simulink library "lib_highLevelController"  (R2025a)
settings: Solver=VariableStepAuto  StartTime=0.0  StopTime=10.0  RelTol=1e-3
settings Model: Creator=Ruben Rodriguez  LastModifiedBy=gordi
settings RTWCC: GPUComputeCapability=3.5

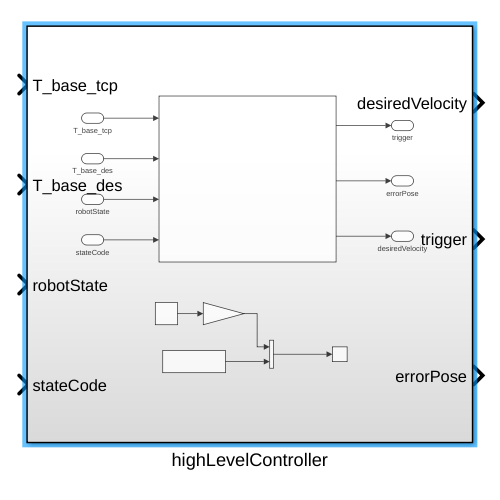
[thumbnail: Simulink's stored preview of the top-level diagram]
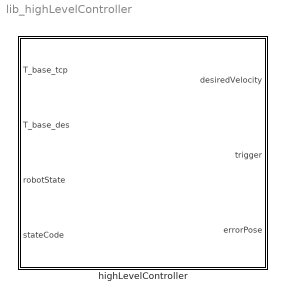
== system lib_highLevelController ==
  highLevelController : Subsystem

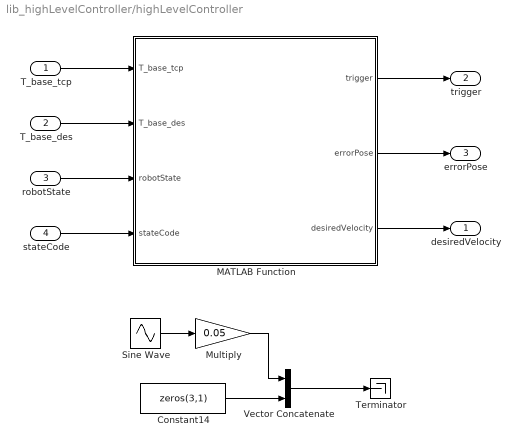
== system lib_highLevelController/highLevelController ==
  T_base_tcp : Inport
  T_base_des : Inport  Port=2
  robotState : Inport  Port=3  OutDataTypeStr=Bus: RobotState
  stateCode : Inport  Port=4
  Constant14 : Constant  Value=zeros(3,1)
  MATLAB Function : MATLAB Function  TreatAsAtomicUnit=on
  Multiply : Gain  Gain=0.05
  Sine Wave : Sin  Amplitude=[1; 1; 1]  SampleTime=0
  Terminator : Terminator
  Vector Concatenate : Concatenate
  desiredVelocity : Outport  OutDataTypeStr=double
  trigger : Outport  Port=2  OutDataTypeStr=double
  errorPose : Outport  Port=3  OutDataTypeStr=double
  wires:
  T_base_tcp/1 -> MATLAB Function/1(T_base_tcp)
  robotState/1 -> MATLAB Function/3(robotState)
  MATLAB Function/3(desiredVelocity) -> desiredVelocity/1
  Vector Concatenate/1 -> Terminator/1
  Sine Wave/1 -> Multiply/1
  Multiply/1 -> Vector Concatenate/1
  Constant14/1 -> Vector Concatenate/2
  T_base_des/1 -> MATLAB Function/2(T_base_des)
  MATLAB Function/1(trigger) -> trigger/1
  stateCode/1 -> MATLAB Function/4(stateCode)
  MATLAB Function/2(errorPose) -> errorPose/1

== matlab function lib_highLevelController/highLevelController/MATLAB Function ==
  data: trigger output; errorPose output; T_base_tcp input size=[4 4]; T_base_des input size=[4 4]; desiredVelocity output size=[6 1]; robotState input Bus: RobotState size=1; stateCode input
function [trigger, errorPose, desiredVelocity] = highLevelController(T_base_tcp, T_base_des, robotState, stateCode)
    [trigger, errorPose, desiredVelocity]  = fun_highLevelController(T_base_tcp, T_base_des, robotState, stateCode);
